simulink model "spherical_wrist"  (R2024b)
settings: Solver=ode23t  StartTime=0.0  StopTime=100  FixedStep=0.001  RelTol=1e-3
InitFcn:
  | WRIST_mk2_1_DataFile
model workspace (MAT data in the model file):
  Damp = Simulink.Parameter
  Damp.Value = 0.0001
  Damp.Complexity = 'real'
  Damp.Dimensions = [1 1]
  Damp.DataType = 'auto'
  Dm = Simulink.Parameter
  Dm.Value = 7.4e-05
  Dm.Complexity = 'real'
  Dm.Dimensions = [1 1]
  Dm.DataType = 'auto'
  Dm.DocUnits = 'mN*m/rpm'
  Jm = Simulink.Parameter
  Jm.Value = 3.3
  Jm.Complexity = 'real'
  Jm.Dimensions = [1 1]
  Jm.DataType = 'auto'
  Jm.DocUnits = 'g*cm^2'
  Km = Simulink.Parameter
  Km.Value = 32.2
  Km.Complexity = 'real'
  Km.Dimensions = [1 1]
  Km.DataType = 'auto'
  Km.DocUnits = 'mN*m/A'
  Tc = Simulink.Parameter
  Tc.Value = 0.001
  Tc.Complexity = 'real'
  Tc.Dimensions = [1 1]
  Tc.DataType = 'auto'
  Tc.DocUnits = 's'
undefined symbols (not defined in the file or in its folder): smiData, X, Y, Z
libraries: sm_lib x370, nesl_utility x32, fl_lib x15, sdl_lib x9, simulink_extras x4, sharedtransform x2, slpidlib x1
(part 1 of 10)
settings Model: Creator=ascalzo  LastModifiedBy=ggandolfi
settings SolverCC: AlgebraicLoopSolver=TrustRegion
settings OptimizationCC: DefaultParameterBehavior=Inlined  UseDivisionForNetSlopeComputation=on  GainParamInheritBuiltInType=on  UseFloatMulNetSlope=on  InlineInvariantSignals=on  ReuseModelBlockBuffer=off  PassReuseOutputArgsAs=Individual arguments  ZeroExternalMemoryAtStartup=off  ZeroInternalMemoryAtStartup=off  NoFixptDivByZeroProtection=on  EfficientFloat2IntCast=on  LifeSpan=1  OptimizeBlockOrder=speed  DifferentSizesBufferReuse=on  EfficientTunableParamExpr=on
settings DebuggingCC: ParameterTunabilityLossMsg=error  UnconnectedInputMsg=warning  UnconnectedOutputMsg=warning  UnconnectedLineMsg=warning
settings HardwareCC: ProdBitPerPointer=32  ProdBitPerSizeT=32  ProdBitPerPtrDiffT=32  ProdLargestAtomicInteger=Long  ProdLargestAtomicFloat=Double  ProdWordSize=32  ProdLongLongMode=on  ProdHWDeviceType=ARM Compatible->ARM Cortex-M
settings ModelReferenceCC: EnableRefExpFcnMdlSchedulingChecks=on
settings SFSimCC: MATLABDynamicMemAlloc=off  SimTargetLang=C++
settings RTWCC: Description=Embedded Coder  SystemTargetFile=ert.tlc  GenCodeOnly=on  PackageGeneratedCodeAndArtifacts=on  PackageName=WristDecoupler.zip  TemplateMakefile=ert_default_tmf  GenerateReport=on  Toolchain=Microsoft Visual C++ 2019 v16.0 | nmake (64-bit Windows)  LaunchReport=on  TargetLang=C++  GPUComputeCapability=3.5  DLArmComputeVersion=19.05
settings CodeAppCC: ForceParamTrailComments=on  IgnoreCustomStorageClasses=off  OperatorAnnotations=on  SimulinkDataObjDesc=on  SFDataObjDesc=on  CustomSymbolStrGlobalVar=rt$N$M  CustomSymbolStrType=$N$M  CustomSymbolStrFcn=$N$M$F  CustomSymbolStrMacro=$N$M  InsertBlockDesc=on  MATLABSourceComments=on
settings ERTTargetCC: TargetLangStandard=C++03 (ISO)  CodeReplacementLibrary=ARM Cortex-M  GenerateSampleERTMain=on  IncludeMdlTerminateFcn=off  CombineSignalStateStructs=on  CodeInterfacePackaging=C++ class  SupportComplex=off  SupportNonInlinedSFcns=on  RootIOFormat=Structure reference  ERTCustomFileTemplate=example_file_process.tlc  ERTFilePackagingFormat=CompactWithDataFile  DynamicArrayContainerType=coder::array
settings ExplorerConfigSet: InternalSimMechanicsExplorerSettings="<ExplorerConfiguration><canonicalview>default</canonicalview><AnimationSetting><BasePlaybackSpeed>1.0</BasePlaybackSpeed><PlaybackSpeedFactor>1.0</PlaybackSpeedFactor></AnimationSetting><TilePanel><TileInfo><Tiles Columns=\"1\" Count=\"1\" Rows=\"1\"><Column Weight=\"1\"/><Row Weight=\"1\"/><Tile Height=\"1\" Width=\"1\" X=\"0\" Y=\"0\"/></Tiles></TileInfo><SceneInfo><SceneViewer><BGColor><R>0.60000002384185791</R><G>0.60000002384185791</G><B>0.60000002384185791</B></BGColor><Camera><DoPerspective>off</DoPerspective><Position><X>0.0033984500914812088</X><Y>-0.99869239330291748</Y><Z>0.0656507387757305771</Z></Position><Center><X>0.0033984500914812088</X><Y>0.00130760669708251953</Y><Z>0.0656507387757305771</Z></Center><Up><X>0</X><Y>-0</Y><Z>1</Z></Up><ViewLimDist>1</ViewLimDist><YLim>0.0676202609390020443</YLim><XLim>0.0894397856975411715</XLim></Camera></SceneViewer></SceneInfo></TilePanel><MechEditorPanel><Cameras/><GfxPanelCameraMap/><VideoCreator><PlaybackSpeedRatio>1.0</PlaybackSpeedRatio><FrameRate>30</FrameRate><VideoFormat>MPEG-4</VideoFormat><FrameSize>[400 400]</FrameSize></VideoCreator></MechEditorPanel></ExplorerConfiguration>"

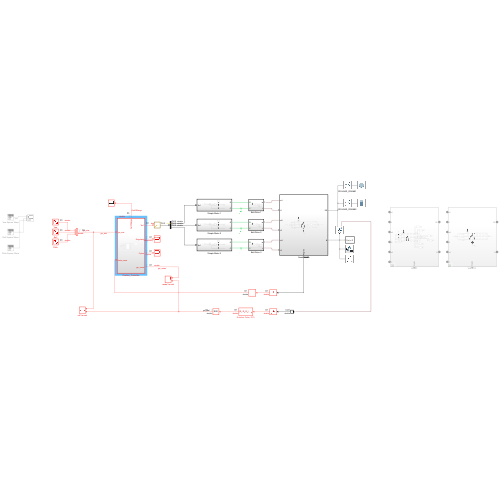
[thumbnail: Simulink's stored preview of the top-level diagram]
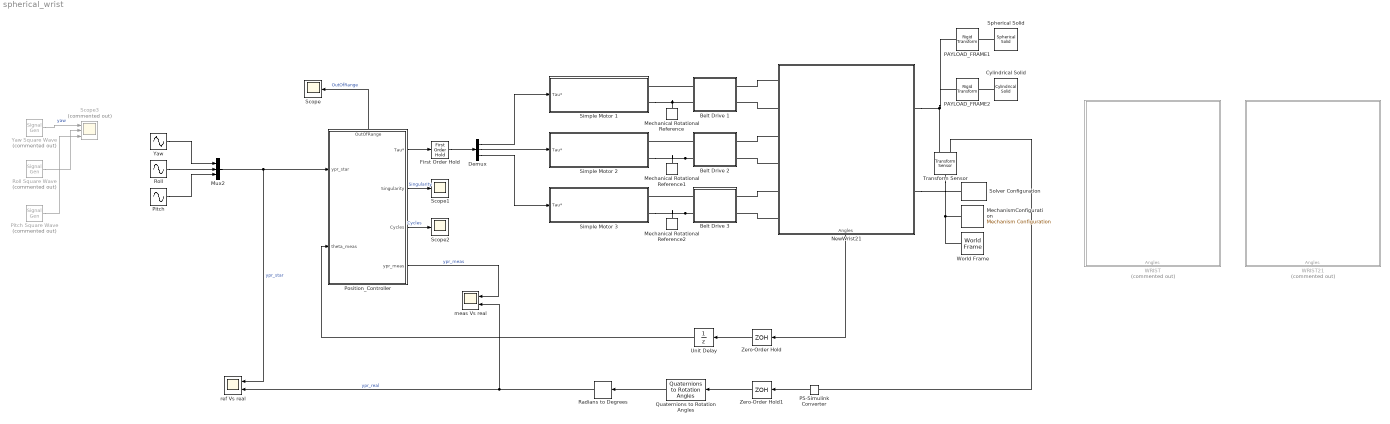
== system spherical_wrist ==
  Belt Drive 1 : Subsystem
  Belt Drive 2 : Subsystem
  Belt Drive 3 : Subsystem
  Cylindrical Solid : sm_lib/Body Elements/Cylindrical Solid  CylinderRadius=4  CylinderRadiusUnits=mm  CylinderLength=56  CylinderLengthUnits=mm  ExportEntireGeometry=off  InertiaType=PointMass  BasedOnType=Density  Density=1000  DensityUnits=kg/m^3  Mass=500  MassUnits=g  CenterOfMass=[0 0 0]  CenterOfMassUnits=m  MomentsOfInertia=[1 1 1]  MomentsOfInertiaUnits=kg*m^2  ProductsOfInertia=[0 0 0]  ProductsOfInertiaUnits=kg*m^2  GraphicType=FromGeometry  MarkerShape=Sphere  MarkerSize=10  GraphicVisPropType=SimpleVisualProperties  GraphicDiffuseColor=[0.5 0.5 0.5]  GraphicOpacity=1  GraphicSpecularColor=[0.5 0.5 0.5 1.0]  GraphicAmbientColor=[0.15 0.15 0.15 1.0]  GraphicEmissiveColor=[0.0 0.0 0.0 1.0]  GraphicShininess=75  DoExposeReferenceFrame=on  SerializedFrames=<Frames/>
  Demux : Demux  Outputs=3
  First Order Hold : FirstOrderHold  ErrorTolerance=inf
  Mechanical Rotational Reference : fl_lib/Mechanical/Rotational Elements/Mechanical Rotational Reference
  Mechanical Rotational Reference1 : fl_lib/Mechanical/Rotational Elements/Mechanical Rotational Reference
  Mechanical Rotational Reference2 : fl_lib/Mechanical/Rotational Elements/Mechanical Rotational Reference
  MechanismConfiguration : sm_lib/Utilities/Mechanism Configuration  UniformGravity=Constant  GravityVector=[0 0 9.80665]  GravityVectorUnits=m/s^2  LinearizationDelta=0.001  JointModeTransitionNonlinearIterations=2
  Mux2 : Mux  Inputs=3
  NewWrist21 : Subsystem
      settings: PortSchema="{\"entries\":[{\"content\":{\"sides\":[{\"content\":{\"connectorIds\":[\"LConn1\",\"LConn2\",\"LConn3\",\"LConn4\",\"LConn5\",\"LConn6\"]},\"type\":\"ConnectorPlacement.EquallySpacedRectSide\",\"uuid\":\"23542f05-d98c-4fd7-a6bd-966b6072cfaf\"},{\"content\":{\"connectorIds\":[\"RConn1\",\"RConn2\"],\"side\":\"RIGHT\"},\"type\":\"ConnectorPlacement.EquallySpacedRectSide\",\"uuid\":\"e7346707-937e-4bb1-b7f6-96a951a5db8c\"},{\"content\":{\"side\":\"TOP\"},\"type\":\"ConnectorPlacement.EquallySpacedRectSide\",\"uuid\":\"63537306-39d7-417a-861f-d22306f14706\"},{\"content\":{\"connectorIds\":[\"Out1\"],\"side\":\"BOTTOM\"},\"type\":\"ConnectorPlacement.EquallySpacedRectSide\",\"uuid\":\"1fb10e15-83ff-4141-85cb-26f173a4368b\"}]},\"type\":\"ConnectorPlacement.EquallySpacedConnector\",\"uuid\":\"ffc830b1-00d2-4766-ad91-ccb75b558bf0\"}],\"packageUris\":[\"http://schema.mathworks.com/mf0/Connector/R2020b\"],\"version\":\"1.0\"}"
  PAYLOAD_FRAME1 : sm_lib/Frames and Transforms/Rigid Transform  RotationMethod=None  FollAlignAxisA=+X  BaseAlignAxisA=+Y  FollAlignAxisB=+Y  BaseAlignAxisB=+Z  RotationStandardAxis=+Z  RotationAngle=smiData.RigidTransform(2).angle  RotationAngleUnits=rad  RotationArbitraryAxis=smiData.RigidTransform(2).axis  RotationSequenceAxes=FollowerAxes  RotationSequence=XYX  RotationSequenceAngles=[0 0 0]  RotationSequenceAnglesUnits=deg  RotationMatrix=[1 0 0; 0 1 0; 0 0 1]  Quaternion=[1 0 0 0]  TranslationMethod=Cartesian  TranslationCartesianOffset=[0 0 70]  TranslationCartesianOffsetUnits=mm  TranslationStandardAxis=+Z  TranslationStandardOffset=0  TranslationStandardOffsetUnits=mm  TranslationROffset=0  TranslationROffsetUnits=m  TranslationThetaOffset=0  TranslationThetaOffsetUnits=deg  TranslationZOffset=0  TranslationZOffsetUnits=m
  PAYLOAD_FRAME2 : sm_lib/Frames and Transforms/Rigid Transform  RotationMethod=None  FollAlignAxisA=+X  BaseAlignAxisA=+Y  FollAlignAxisB=+Y  BaseAlignAxisB=+Z  RotationStandardAxis=+Z  RotationAngle=smiData.RigidTransform(2).angle  RotationAngleUnits=rad  RotationArbitraryAxis=smiData.RigidTransform(2).axis  RotationSequenceAxes=FollowerAxes  RotationSequence=XYX  RotationSequenceAngles=[0 0 0]  RotationSequenceAnglesUnits=deg  RotationMatrix=[1 0 0; 0 1 0; 0 0 1]  Quaternion=[1 0 0 0]  TranslationMethod=Cartesian  TranslationCartesianOffset=[0 0 30]  TranslationCartesianOffsetUnits=mm  TranslationStandardAxis=+Z  TranslationStandardOffset=0  TranslationStandardOffsetUnits=mm  TranslationROffset=0  TranslationROffsetUnits=m  TranslationThetaOffset=0  TranslationThetaOffsetUnits=deg  TranslationZOffset=0  TranslationZOffsetUnits=m
  PS-Simulink Converter : nesl_utility/PS-Simulink Converter  PhysicalDomain=network_engine_domain  SubClassName=ps_output  LeftPortType=input  RightPortType=output  PseudoPeriodic=off  Frequencies=[]  VectorFormat=1-D array  Unit=inherit  AffineConversion=off
  Pitch : Sin  Amplitude=20  Frequency=2*pi/10  SampleTime=Tc
  Pitch Square Wave : SignalGenerator  Commented=on  WaveForm=square  Amplitude=75  Frequency=2*pi/10  Units=rad/sec
  Position_Controller : Subsystem  TreatAsAtomicUnit=on  SystemSampleTime=0.001
      settings: MinAlgLoopOccurrences=on  PortSchema="{\"entries\":[{\"content\":{\"sides\":[{\"content\":{\"connectorIds\":[\"In1\",\"In2\"]},\"type\":\"ConnectorPlacement.EquallySpacedRectSide\",\"uuid\":\"83213a6a-d539-4d4b-893d-998d212c9f51\"},{\"content\":{\"connectorIds\":[\"Out1\",\"Out2\",\"Out3\",\"Out4\"],\"side\":\"RIGHT\"},\"type\":\"ConnectorPlacement.EquallySpacedRectSide\",\"uuid\":\"07d19463-f1b8-4ef2-82ae-a356a5259b0c\"},{\"content\":{\"connectorIds\":[\"Out5\"],\"side\":\"TOP\"},\"type\":\"ConnectorPlacement.EquallySpacedRectSide\",\"uuid\":\"262960f5-5579-40eb-9028-5284e67b897c\"}]},\"type\":\"ConnectorPlacement.EquallySpacedConnector\",\"uuid\":\"3a54d725-4b36-4299-8af9-8f83752d9c8a\"}],\"packageUris\":[\"http://schema.mathworks.com/mf0/Connector/R2020b\"],\"version\":\"1.0\"}"
  Quaternions to Rotation Angles : sharedtransform/Quaternions to Rotation Angles  rotationOrder=ZYX  aMode=aMode
  Radians to Degrees : simulink_extras/Transformations/Radians to Degrees
  Roll : Sin  Amplitude=33  Frequency=(1+sqrt(5))  SampleTime=Tc
  Roll Square Wave : SignalGenerator  Commented=on  WaveForm=square  Amplitude=75  Frequency=(1+sqrt(5))  Units=rad/sec
  Scope : Scope
  Scope1 : Scope
  Scope2 : Scope
  Scope3 : Scope  Commented=on  NumInputPorts=3
  Simple Motor 1 : Subsystem
  Simple Motor 2 : Subsystem
  Simple Motor 3 : Subsystem
  Solver Configuration : nesl_utility/Solver Configuration  PhysicalDomain=network_engine_domain  SubClassName=solver  LeftPortType=input  RightPortType=generic  Tones=[]  Harmonics=[]  SimulateNoise=off  Profile=off  UseLocalSampling=off  EnableSwitchedLinearOptims=on  FrequencyDomain=off  UseCCode=off  RelTol=0.001  AbsTol=1e-06  MinStep=1e-09  ToWorkspace=off  RevertToSquareIcSolve=off  NumHomotopyIterations=100  PhasorMode=off  PhasorModeNumHarmonics=1  ConsistencySolver=NEWTON_FTOL  IndexReductionMethod=DerivativeReplacement  DoDC=off  ResidualTolerance=1e-09  ConsistencyTolSource=GLOBAL  ConsistencyAbsTol=0.001  ConsistencyRelTol=0.001  ConsistencyTolFactor=0.001  UseLocalSolver=off  LocalSolverChoice=NE_TRAPEZOIDAL_ADVANCER  ResolveIndetEquations=on  FunctionEvalNumThread=1  LocalSolverSampleTime=0.0001  DoFixedCost=off  MaxNonlinIter=3  MaxModeIter=2  ComputeImpulses=off  ImpulseIterations=2  LinearAlgebra=auto  LinearAlgebraNumThread=0  EquationFormulation=NE_TIME_EF  DelaysMemoryBudget=1024  AutomaticFiltering=on  FilteringTimeConstant=0.001  PartitionStorageMethod=AS_NEEDED  PartitionMemoryBudget=1024  PartitionMethod=ROBUST  MultibodyUseLocalSolver=off  MultibodyLocalSolverChoice=ODE1  MultibodyLocalSolverSampleTime=0.001
  Spherical Solid : sm_lib/Body Elements/Spherical Solid  SphereRadius=15  SphereRadiusUnits=mm  ExportEntireGeometry=off  InertiaType=CalculateFromGeometry  BasedOnType=Density  Density=1000  DensityUnits=kg/m^3  Mass=1  MassUnits=kg  CenterOfMass=[0 0 0]  CenterOfMassUnits=m  MomentsOfInertia=[1 1 1]  MomentsOfInertiaUnits=kg*m^2  ProductsOfInertia=[0 0 0]  ProductsOfInertiaUnits=kg*m^2  GraphicType=FromGeometry  MarkerShape=Sphere  MarkerSize=10  GraphicVisPropType=SimpleVisualProperties  GraphicDiffuseColor=[0.5 0.5 0.5]  GraphicOpacity=1.0  GraphicSpecularColor=[0.5 0.5 0.5 1.0]  GraphicAmbientColor=[0.15 0.15 0.15 1.0]  GraphicEmissiveColor=[0.0 0.0 0.0 1.0]  GraphicShininess=75  DoExposeReferenceFrame=on  SerializedFrames=<Frames/>
  Transform Sensor : sm_lib/Frames and Transforms/Transform Sensor  MeasurementFrame=World  RotationSequence=XYX  SenseAngle=off  SenseAxis=off  SenseQ=on  SenseR=off  SenseRotationSequence=off  SenseOmegaX=off  SenseOmegaY=off  SenseOmegaZ=off  SenseOmega=off  SenseQDot=off  SenseRDot=off  SenseRotationSequenceDot=off  SenseAlphaX=off  SenseAlphaY=off  SenseAlphaZ=off  SenseAlpha=off  SenseQDDot=off  SenseRDDot=off  SenseX=off  SenseY=off  SenseZ=off  SenseXYZ=off  SenseRad=off  SenseAzim=off  SenseDist=off  SenseInc=off  SenseXDot=off  SenseYDot=off  SenseZDot=off  SenseXYZDot=off  SenseRadDot=off  SenseAzimDot=off  SenseDistDot=off  SenseIncDot=off  SenseXDDot=off  SenseYDDot=off  SenseZDDot=off  SenseXYZDDot=off  SenseRadDDot=off  SenseAzimDDot=off  SenseDistDDot=off  SenseIncDDot=off
  Unit Delay : UnitDelay  SampleTime=-1  HasFrameUpgradeWarning=on
  WRIST : Subsystem  Commented=on
      settings: PortSchema="{\"entries\":[{\"content\":{\"sides\":[{\"content\":{\"connectorIds\":[\"LConn1\",\"LConn2\",\"LConn3\",\"LConn4\",\"LConn5\",\"LConn6\"]},\"type\":\"ConnectorPlacement.EquallySpacedRectSide\",\"uuid\":\"837cba77-e4d8-410a-871c-09f9d5b58985\"},{\"content\":{\"connectorIds\":[\"RConn1\",\"RConn2\"],\"side\":\"RIGHT\"},\"type\":\"ConnectorPlacement.EquallySpacedRectSide\",\"uuid\":\"e99e27fa-5cde-4df4-999c-5c540dbd874f\"},{\"content\":{\"connectorIds\":[],\"side\":\"TOP\"},\"type\":\"ConnectorPlacement.EquallySpacedRectSide\",\"uuid\":\"93dbe70b-6d44-4b10-9b14-70f8e934205d\"},{\"content\":{\"connectorIds\":[\"Out1\"],\"side\":\"BOTTOM\"},\"type\":\"ConnectorPlacement.EquallySpacedRectSide\",\"uuid\":\"bafba6b5-af66-4d82-b4b8-19931a0ab184\"}]},\"type\":\"ConnectorPlacement.EquallySpacedConnector\",\"uuid\":\"c57b24f6-44a7-49b3-8fbc-a4c709c10c31\"}],\"packageUris\":[\"http://schema.mathworks.com/mf0/Connector/19700101\"],\"version\":\"1.0\"}"
  WRIST21 : Subsystem  Commented=on
      settings: PortSchema="{\"entries\":[{\"content\":{\"sides\":[{\"content\":{\"connectorIds\":[\"LConn1\",\"LConn2\",\"LConn3\",\"LConn4\",\"LConn5\",\"LConn6\"]},\"type\":\"ConnectorPlacement.EquallySpacedRectSide\",\"uuid\":\"837cba77-e4d8-410a-871c-09f9d5b58985\"},{\"content\":{\"connectorIds\":[\"RConn1\",\"RConn2\"],\"side\":\"RIGHT\"},\"type\":\"ConnectorPlacement.EquallySpacedRectSide\",\"uuid\":\"e99e27fa-5cde-4df4-999c-5c540dbd874f\"},{\"content\":{\"side\":\"TOP\"},\"type\":\"ConnectorPlacement.EquallySpacedRectSide\",\"uuid\":\"93dbe70b-6d44-4b10-9b14-70f8e934205d\"},{\"content\":{\"connectorIds\":[\"Out1\"],\"side\":\"BOTTOM\"},\"type\":\"ConnectorPlacement.EquallySpacedRectSide\",\"uuid\":\"bafba6b5-af66-4d82-b4b8-19931a0ab184\"}]},\"type\":\"ConnectorPlacement.EquallySpacedConnector\",\"uuid\":\"c57b24f6-44a7-49b3-8fbc-a4c709c10c31\"}],\"packageUris\":[\"http://schema.mathworks.com/mf0/Connector/R2020b\"],\"version\":\"1.0\"}"
  World Frame : sm_lib/Frames and Transforms/World Frame
  Yaw : Sin  Amplitude=92  Frequency=2*pi/40  SampleTime=Tc
  Yaw Square Wave : SignalGenerator  Commented=on  WaveForm=square  Amplitude=90  Frequency=2*pi/40  Units=rad/sec
  Zero-Order Hold : ZeroOrderHold  SampleTime=Tc
  Zero-Order Hold1 : ZeroOrderHold  SampleTime=Tc
  meas Vs real : Scope  NumInputPorts=2
  ref Vs real : Scope  NumInputPorts=2
  wires:
  NewWrist21/1(Angles) -> Zero-Order Hold/1
  Radians to Degrees/1 -> meas Vs real/2, ref Vs real/2  "ypr_real"
  PS-Simulink Converter/1 -> Zero-Order Hold1/1
  Quaternions to Rotation Angles/1 -> Radians to Degrees/1
  Mux2/1 -> Position_Controller/1(ypr_star), ref Vs real/1  "ypr_star"
  Demux/1 -> Simple Motor 1/1(Tau*)
  Demux/2 -> Simple Motor 2/1(Tau*)
  Demux/3 -> Simple Motor 3/1(Tau*)
  First Order Hold/1 -> Demux/1
  Position_Controller/4(ypr_meas) -> meas Vs real/1  "ypr_meas"
  Position_Controller/1(Tau*) -> First Order Hold/1
  Position_Controller/3(Cycles) -> Scope2/1  "Cycles"
  Position_Controller/2(Singularity) -> Scope1/1  "Singularity"
  Zero-Order Hold1/1 -> Quaternions to Rotation Angles/1
  Position_Controller/5(OutOfRange) -> Scope/1  "OutOfRange"
  Zero-Order Hold/1 -> Unit Delay/1
  Roll Square Wave/1 -> Scope3/2
  Pitch Square Wave/1 -> Scope3/3
  Yaw Square Wave/1 -> Scope3/1  "yaw"
  Yaw/1 -> Mux2/1
  Roll/1 -> Mux2/2
  Pitch/1 -> Mux2/3
  Unit Delay/1 -> Position_Controller/2(theta_meas)
  connections:
  World Frame/RConn1 -- NewWrist21/RConn2 -- Transform Sensor/LConn1 -- Solver Configuration/RConn1 -- MechanismConfiguration/RConn1
  PAYLOAD_FRAME1/LConn1 -- PAYLOAD_FRAME2/LConn1 -- NewWrist21/RConn1 -- Transform Sensor/RConn1
  Transform Sensor/RConn2 -- PS-Simulink Converter/LConn1
  Cylindrical Solid/RConn1 -- PAYLOAD_FRAME2/RConn1
  Spherical Solid/RConn1 -- PAYLOAD_FRAME1/RConn1
  NewWrist21/LConn1 -- Belt Drive 1/RConn1
  Mechanical Rotational Reference/LConn1 -- Simple Motor 1/RConn2 -- Belt Drive 1/LConn2
  Belt Drive 1/LConn1 -- Simple Motor 1/RConn1
  Belt Drive 2/LConn2 -- Simple Motor 2/RConn2 -- Mechanical Rotational Reference1/LConn1
  Belt Drive 2/LConn1 -- Simple Motor 2/RConn1
  NewWrist21/LConn3 -- Belt Drive 2/RConn1
  Belt Drive 3/LConn2 -- Simple Motor 3/RConn2 -- Mechanical Rotational Reference2/LConn1
  Belt Drive 3/LConn1 -- Simple Motor 3/RConn1
  NewWrist21/LConn5 -- Belt Drive 3/RConn1
  NewWrist21/LConn2 -- Belt Drive 1/RConn2
  NewWrist21/LConn4 -- Belt Drive 2/RConn2
  NewWrist21/LConn6 -- Belt Drive 3/RConn2

== system spherical_wrist/Belt Drive 1 ==
  Belt Drive : sdl_lib/Couplings & Drives/Belt Drive  drive_type=sdl.enum.wrap_configuration.open  belt_type=sdl.enum.belt_type.ideal  sheave_ang=30 deg  num_belts=1  model_f_c=sdl.enum.model_centrifugal.off  linear_density=0.6 kg/m  model_compliance=sdl.enum.compliance.off  stiffness=1e4 N/m  damping=1e3 N/(m/s)  tension=100 N  breakable=sdl.enum.max_tension.off  F_max=1e5 N  r_pulley_A=14 mm  b_pulley_A=0.1 N*m/(rad/s)  model_inertia_A=sdl.enum.model_inertia.on  pulley_inertia_A=10 g*mm^2  initial_velocity_A=0 rad/s  r_pulley_B=28 mm  b_pulley_B=0.1 N*m/(rad/s)  model_inertia_B=sdl.enum.model_inertia.on  pulley_inertia_B=10 g*mm^2  initial_velocity_B=0 rad/s  friction_model=sdl.enum.PulleyModel.Continuous  initial_state_locked_A=sdl.enum.initial_lock.unlocked  initial_state_locked_B=sdl.enum.initial_lock.unlocked  mu=0.5  mu_static=0.5  mu_kinetic=0.42  wrap_parameterization=sdl.enum.wrap_parameterization.centers  d_centers=0.5 m  phi_wrap_A=145 deg  phi_wrap_B=215 deg  v_thr=0.001 m/s  f_thr=1 N
      settings: InternalSimscapePortConfiguration="{\"Bottom\":[],\"Left\":[{\"id\":\"A\",\"label\":\"A\",\"type\":\"foundation.mechanical.rotational.rotational\"}],\"Right\":[{\"id\":\"B\",\"label\":\"B\",\"type\":\"foundation.mechanical.rotational.rotational\"}],\"Top\":[]}"
  Inertia1 : fl_lib/Mechanical/Rotational Elements/Inertia  inertia=34 g*mm^2  num_ports=foundation.enum.numPorts2.one  w_specify=off  w_priority=High  w=0 rad/s  w_nominal_specify=off  w_nominal_value=1  w_nominal_unit=rad/s  t_specify=off  t_priority=None  t=0 N*m  t_nominal_specify=off  t_nominal_value=1  t_nominal_unit=N*m
  Rotational Multibody Interface : fl_lib/Mechanical/Multibody Interfaces/Rotational Multibody Interface
  Simple Gear : sdl_lib/Gears/Simple Gear  ratio=196  rotation_direction=3-2*(1)  friction_model=sdl.enum.gear_efficiencies_load.constant  T_noload=0.1 N*m  T_nom=5 N*m  efficiency_nom=0.8  efficiency=0.78  temperature_TLU=[280, 300, 320] K  load_TLU=[1, 5, 10] N*m  efficiency_TLU=[.95, .9, .85]  efficiency_TLU2=[.85, .8, .75; .95, .9, .85; .85, .8, .7]  w_thr=0.01 rad/s  pwr_thr=9 W  enable_backlash=false  hardstop_model=simscape.enum.hardstop.smooth  backlash_distance=1e-3 mm  r_base=0.1 m  transition=1e-4 mm  backlash_stiffness=1e7 N/m  backlash_damping=1e6 N*s/m  coeff_rest=0  v_tol=0.001 m/s  f_tol=0 N  mu_visc=[0, 0] N*m/(rad/s)  thermal_mass=50 J/K  temperature_specify=off  temperature_priority=High  temperature=300 K  temperature_nominal_specify=off  temperature_nominal_value=1  temperature_nominal_unit=K  x_backlash_specify=off  x_backlash_priority=None  x_backlash=0 mm  x_backlash_nominal_specify=off  x_backlash_nominal_value=1  x_backlash_nominal_unit=mm  f_hardstop_specify=off  f_hardstop_priority=None  f_hardstop=0 N  f_hardstop_nominal_specify=off  f_hardstop_nominal_value=1  f_hardstop_nominal_unit=N  v_backlash_specify=off  v_backlash_priority=None  v_backlash=0 m/s  v_backlash_nominal_specify=off  v_backlash_nominal_value=1  v_backlash_nominal_unit=m/s
  R : PMIOPort  Side=Left
  C : PMIOPort  Port=2  Side=Left
  w : PMIOPort  Port=3  Side=Right
  t : PMIOPort  Port=4  Side=Right
  connections:
  Rotational Multibody Interface/RConn2 -- Belt Drive/RConn1
  Simple Gear/LConn1 -- R/RConn1 -- Inertia1/LConn1
  Rotational Multibody Interface/RConn1 -- w/RConn1
  Belt Drive/LConn1 -- Simple Gear/RConn1
  Rotational Multibody Interface/LConn1 -- t/RConn1
  Rotational Multibody Interface/LConn2 -- C/RConn1

== system spherical_wrist/Belt Drive 2 ==
  Belt Drive : sdl_lib/Couplings & Drives/Belt Drive  drive_type=sdl.enum.wrap_configuration.open  belt_type=sdl.enum.belt_type.ideal  sheave_ang=30 deg  num_belts=1  model_f_c=sdl.enum.model_centrifugal.off  linear_density=0.6 kg/m  model_compliance=sdl.enum.compliance.off  stiffness=1e4 N/m  damping=1e3 N/(m/s)  tension=100 N  breakable=sdl.enum.max_tension.off  F_max=1e5 N  r_pulley_A=14 mm  b_pulley_A=0.1 N*m/(rad/s)  model_inertia_A=sdl.enum.model_inertia.on  pulley_inertia_A=10 g*mm^2  initial_velocity_A=0 rad/s  r_pulley_B=28 mm  b_pulley_B=0.1 N*m/(rad/s)  model_inertia_B=sdl.enum.model_inertia.on  pulley_inertia_B=10 g*mm^2  initial_velocity_B=0 rad/s  friction_model=sdl.enum.PulleyModel.Continuous  initial_state_locked_A=sdl.enum.initial_lock.unlocked  initial_state_locked_B=sdl.enum.initial_lock.unlocked  mu=0.5  mu_static=0.5  mu_kinetic=0.42  wrap_parameterization=sdl.enum.wrap_parameterization.centers  d_centers=0.5 m  phi_wrap_A=145 deg  phi_wrap_B=215 deg  v_thr=0.001 m/s  f_thr=1 N
      settings: InternalSimscapePortConfiguration="{\"Bottom\":[],\"Left\":[{\"id\":\"A\",\"label\":\"A\",\"type\":\"foundation.mechanical.rotational.rotational\"}],\"Right\":[{\"id\":\"B\",\"label\":\"B\",\"type\":\"foundation.mechanical.rotational.rotational\"}],\"Top\":[]}"
  Inertia1 : fl_lib/Mechanical/Rotational Elements/Inertia  inertia=34 g*mm^2  num_ports=foundation.enum.numPorts2.one  w_specify=off  w_priority=High  w=0 rad/s  w_nominal_specify=off  w_nominal_value=1  w_nominal_unit=rad/s  t_specify=off  t_priority=None  t=0 N*m  t_nominal_specify=off  t_nominal_value=1  t_nominal_unit=N*m
  Rotational Multibody Interface : fl_lib/Mechanical/Multibody Interfaces/Rotational Multibody Interface
  Simple Gear : sdl_lib/Gears/Simple Gear  ratio=196  rotation_direction=3-2*(1)  friction_model=sdl.enum.gear_efficiencies_load.constant  T_noload=0.1 N*m  T_nom=5 N*m  efficiency_nom=0.8  efficiency=0.78  temperature_TLU=[280, 300, 320] K  load_TLU=[1, 5, 10] N*m  efficiency_TLU=[.95, .9, .85]  efficiency_TLU2=[.85, .8, .75; .95, .9, .85; .85, .8, .7]  w_thr=0.01 rad/s  pwr_thr=9 W  enable_backlash=false  hardstop_model=simscape.enum.hardstop.smooth  backlash_distance=1e-3 mm  r_base=0.1 m  transition=1e-4 mm  backlash_stiffness=1e7 N/m  backlash_damping=1e6 N*s/m  coeff_rest=0  v_tol=0.001 m/s  f_tol=0 N  mu_visc=[0, 0] N*m/(rad/s)  thermal_mass=50 J/K  temperature_specify=off  temperature_priority=High  temperature=300 K  temperature_nominal_specify=off  temperature_nominal_value=1  temperature_nominal_unit=K  x_backlash_specify=off  x_backlash_priority=None  x_backlash=0 mm  x_backlash_nominal_specify=off  x_backlash_nominal_value=1  x_backlash_nominal_unit=mm  f_hardstop_specify=off  f_hardstop_priority=None  f_hardstop=0 N  f_hardstop_nominal_specify=off  f_hardstop_nominal_value=1  f_hardstop_nominal_unit=N  v_backlash_specify=off  v_backlash_priority=None  v_backlash=0 m/s  v_backlash_nominal_specify=off  v_backlash_nominal_value=1  v_backlash_nominal_unit=m/s
  R : PMIOPort  Side=Left
  C : PMIOPort  Port=2  Side=Left
  w : PMIOPort  Port=3  Side=Right
  t : PMIOPort  Port=4  Side=Right
  connections:
  Rotational Multibody Interface/RConn2 -- Belt Drive/RConn1
  Inertia1/LConn1 -- Simple Gear/LConn1 -- R/RConn1
  Rotational Multibody Interface/RConn1 -- w/RConn1
  Belt Drive/LConn1 -- Simple Gear/RConn1
  Rotational Multibody Interface/LConn1 -- t/RConn1
  Rotational Multibody Interface/LConn2 -- C/RConn1

== system spherical_wrist/Belt Drive 3 ==
  Belt Drive : sdl_lib/Couplings & Drives/Belt Drive  drive_type=sdl.enum.wrap_configuration.open  belt_type=sdl.enum.belt_type.ideal  sheave_ang=30 deg  num_belts=1  model_f_c=sdl.enum.model_centrifugal.off  linear_density=0.6 kg/m  model_compliance=sdl.enum.compliance.off  stiffness=1e4 N/m  damping=1e3 N/(m/s)  tension=100 N  breakable=sdl.enum.max_tension.off  F_max=1e5 N  r_pulley_A=14 mm  b_pulley_A=0.1 N*m/(rad/s)  model_inertia_A=sdl.enum.model_inertia.on  pulley_inertia_A=10 g*mm^2  initial_velocity_A=0 rad/s  r_pulley_B=28 mm  b_pulley_B=0.1 N*m/(rad/s)  model_inertia_B=sdl.enum.model_inertia.on  pulley_inertia_B=10 g*mm^2  initial_velocity_B=0 rad/s  friction_model=sdl.enum.PulleyModel.Continuous  initial_state_locked_A=sdl.enum.initial_lock.unlocked  initial_state_locked_B=sdl.enum.initial_lock.unlocked  mu=0.5  mu_static=0.5  mu_kinetic=0.42  wrap_parameterization=sdl.enum.wrap_parameterization.centers  d_centers=0.5 m  phi_wrap_A=145 deg  phi_wrap_B=215 deg  v_thr=0.001 m/s  f_thr=1 N
      settings: InternalSimscapePortConfiguration="{\"Bottom\":[],\"Left\":[{\"id\":\"A\",\"label\":\"A\",\"type\":\"foundation.mechanical.rotational.rotational\"}],\"Right\":[{\"id\":\"B\",\"label\":\"B\",\"type\":\"foundation.mechanical.rotational.rotational\"}],\"Top\":[]}"
  Inertia1 : fl_lib/Mechanical/Rotational Elements/Inertia  inertia=34 g*mm^2  num_ports=foundation.enum.numPorts2.one  w_specify=off  w_priority=High  w=0 rad/s  w_nominal_specify=off  w_nominal_value=1  w_nominal_unit=rad/s  t_specify=off  t_priority=None  t=0 N*m  t_nominal_specify=off  t_nominal_value=1  t_nominal_unit=N*m
  Rotational Multibody Interface : fl_lib/Mechanical/Multibody Interfaces/Rotational Multibody Interface
  Simple Gear : sdl_lib/Gears/Simple Gear  ratio=196  rotation_direction=3-2*(1)  friction_model=sdl.enum.gear_efficiencies_load.constant  T_noload=0.1 N*m  T_nom=5 N*m  efficiency_nom=0.8  efficiency=0.78  temperature_TLU=[280, 300, 320] K  load_TLU=[1, 5, 10] N*m  efficiency_TLU=[.95, .9, .85]  efficiency_TLU2=[.85, .8, .75; .95, .9, .85; .85, .8, .7]  w_thr=0.01 rad/s  pwr_thr=9 W  enable_backlash=false  hardstop_model=simscape.enum.hardstop.smooth  backlash_distance=1e-3 mm  r_base=0.1 m  transition=1e-4 mm  backlash_stiffness=1e7 N/m  backlash_damping=1e6 N*s/m  coeff_rest=0  v_tol=0.001 m/s  f_tol=0 N  mu_visc=[0, 0] N*m/(rad/s)  thermal_mass=50 J/K  temperature_specify=off  temperature_priority=High  temperature=300 K  temperature_nominal_specify=off  temperature_nominal_value=1  temperature_nominal_unit=K  x_backlash_specify=off  x_backlash_priority=None  x_backlash=0 mm  x_backlash_nominal_specify=off  x_backlash_nominal_value=1  x_backlash_nominal_unit=mm  f_hardstop_specify=off  f_hardstop_priority=None  f_hardstop=0 N  f_hardstop_nominal_specify=off  f_hardstop_nominal_value=1  f_hardstop_nominal_unit=N  v_backlash_specify=off  v_backlash_priority=None  v_backlash=0 m/s  v_backlash_nominal_specify=off  v_backlash_nominal_value=1  v_backlash_nominal_unit=m/s
  R : PMIOPort  Side=Left
  C : PMIOPort  Port=2  Side=Left
  w : PMIOPort  Port=3  Side=Right
  t : PMIOPort  Port=4  Side=Right
  connections:
  Rotational Multibody Interface/RConn2 -- Belt Drive/RConn1
  Inertia1/LConn1 -- Simple Gear/LConn1 -- R/RConn1
  Rotational Multibody Interface/RConn1 -- w/RConn1
  Belt Drive/LConn1 -- Simple Gear/RConn1
  Rotational Multibody Interface/LConn1 -- t/RConn1
  Rotational Multibody Interface/LConn2 -- C/RConn1

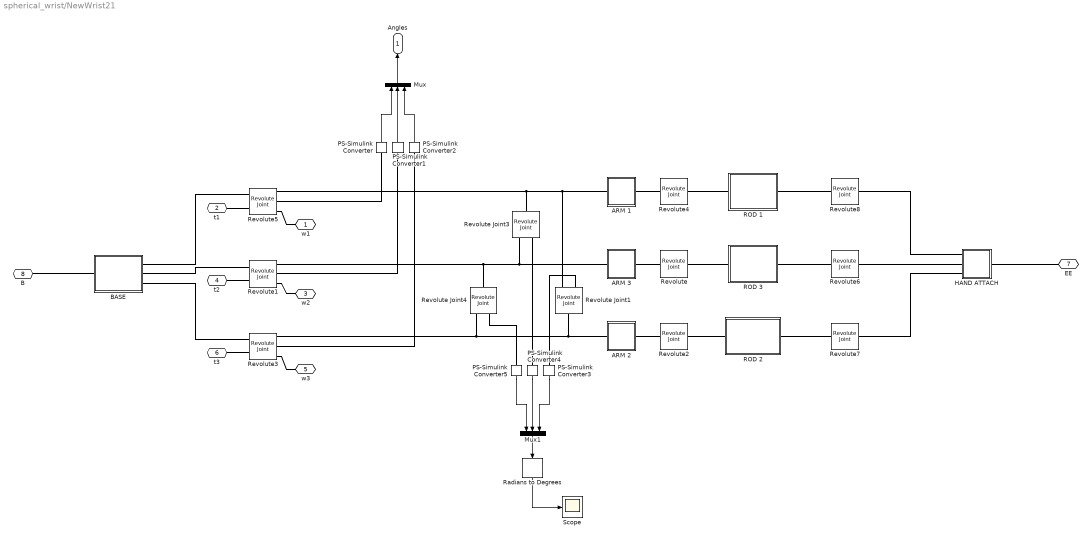
== system spherical_wrist/NewWrist21 ==
  ARM 1 : Subsystem
  ARM 2 : Subsystem
  ARM 3 : Subsystem
  BASE : Subsystem
  HAND ATTACH : Subsystem
  Mux : Mux  Inputs=3
  Mux1 : Mux  Inputs=3
  PS-Simulink Converter : nesl_utility/PS-Simulink Converter  PhysicalDomain=network_engine_domain  SubClassName=ps_output  LeftPortType=input  RightPortType=output  PseudoPeriodic=off  Frequencies=[]  VectorFormat=1-D array  Unit=deg  AffineConversion=off
  PS-Simulink Converter1 : nesl_utility/PS-Simulink Converter  PhysicalDomain=network_engine_domain  SubClassName=ps_output  LeftPortType=input  RightPortType=output  PseudoPeriodic=off  Frequencies=[]  VectorFormat=1-D array  Unit=deg  AffineConversion=off
  PS-Simulink Converter2 : nesl_utility/PS-Simulink Converter  PhysicalDomain=network_engine_domain  SubClassName=ps_output  LeftPortType=input  RightPortType=output  PseudoPeriodic=off  Frequencies=[]  VectorFormat=1-D array  Unit=deg  AffineConversion=off
  PS-Simulink Converter3 : nesl_utility/PS-Simulink Converter  PhysicalDomain=network_engine_domain  SubClassName=ps_output  LeftPortType=input  RightPortType=output  PseudoPeriodic=off  Frequencies=[]  VectorFormat=inherit  Unit=inherit  AffineConversion=off
  PS-Simulink Converter4 : nesl_utility/PS-Simulink Converter  PhysicalDomain=network_engine_domain  SubClassName=ps_output  LeftPortType=input  RightPortType=output  PseudoPeriodic=off  Frequencies=[]  VectorFormat=inherit  Unit=inherit  AffineConversion=off
  PS-Simulink Converter5 : nesl_utility/PS-Simulink Converter  PhysicalDomain=network_engine_domain  SubClassName=ps_output  LeftPortType=input  RightPortType=output  PseudoPeriodic=off  Frequencies=[]  VectorFormat=inherit  Unit=inherit  AffineConversion=off
  ROD 1 : Subsystem
  ROD 2 : Subsystem
  ROD 3 : Subsystem
  Radians to Degrees : simulink_extras/Transformations/Radians to Degrees
  Revolute : sm_lib/Joints/Revolute Joint  JointMode=Normal  CompositeWrenchDir=FollowerOnBase  CompositeWrenchFrame=BaseFrame  SenseConstraintForce=off  SenseConstraintTorque=off  SenseTotalForce=off  SenseTotalTorque=off  PositionTargetSpecify=on  PositionTargetPriority=Low  PositionTargetValue=smiData.RevoluteJoint(1).Rz.Pos  PositionTargetValueUnits=deg  VelocityTargetSpecify=off  VelocityTargetPriority=High  VelocityTargetValue=0  VelocityTargetValueUnits=deg/s  EquilibriumPosition=0  EquilibriumPositionUnits=deg  SpringStiffness=0  SpringStiffnessUnits=N*m/deg  DampingCoefficient=0  DampingCoefficientUnits=N*m/(deg/s)  LowerLimitSpecify=off  LowerLimitBound=-90  LowerLimitBoundUnits=deg  LowerLimitStiffness=1e4  LowerLimitStiffnessUnits=N*m/deg  LowerLimitDamping=10  LowerLimitDampingUnits=N*m/(deg/s)  LowerLimitTransitionRegionWidth=0.1  LowerLimitTransitionRegionWidthUnits=deg  UpperLimitSpecify=off  UpperLimitBound=90  UpperLimitBoundUnits=deg  UpperLimitStiffness=1e4  UpperLimitStiffnessUnits=N*m/deg  UpperLimitDamping=10  UpperLimitDampingUnits=N*m/(deg/s)  UpperLimitTransitionRegionWidth=0.1  UpperLimitTransitionRegionWidthUnits=deg  TorqueActuationMode=NoTorque  MotionActuationMode=ComputedMotion  SensePosition=off  SenseVelocity=off  SenseAcceleration=off  SenseTorqueForce=off  SenseLowerLimitTorqueForce=off  SenseUpperLimitTorqueForce=off
  Revolute Joint1 : sm_lib/Joints/Revolute Joint  JointMode=Normal  CompositeWrenchDir=FollowerOnBase  CompositeWrenchFrame=BaseFrame  SenseConstraintForce=off  SenseConstraintTorque=off  SenseTotalForce=off  SenseTotalTorque=off  PositionTargetSpecify=off  PositionTargetPriority=Low  PositionTargetValue=130  PositionTargetValueUnits=deg  VelocityTargetSpecify=off  VelocityTargetPriority=High  VelocityTargetValue=0  VelocityTargetValueUnits=deg/s  EquilibriumPosition=0  EquilibriumPositionUnits=deg  SpringStiffness=0  SpringStiffnessUnits=N*m/deg  DampingCoefficient=0  DampingCoefficientUnits=N*m/(deg/s)  LowerLimitSpecify=on  LowerLimitBound=33  LowerLimitBoundUnits=deg  LowerLimitStiffness=1e4  LowerLimitStiffnessUnits=N*m/deg  LowerLimitDamping=10  LowerLimitDampingUnits=N*m/(deg/s)  LowerLimitTransitionRegionWidth=0.1  LowerLimitTransitionRegionWidthUnits=deg  UpperLimitSpecify=off  UpperLimitBound=90  UpperLimitBoundUnits=deg  UpperLimitStiffness=1e4  UpperLimitStiffnessUnits=N*m/deg  UpperLimitDamping=10  UpperLimitDampingUnits=N*m/(deg/s)  UpperLimitTransitionRegionWidth=0.1  UpperLimitTransitionRegionWidthUnits=deg  TorqueActuationMode=NoTorque  MotionActuationMode=ComputedMotion  SensePosition=on  SenseVelocity=off  SenseAcceleration=off  SenseTorqueForce=off  SenseLowerLimitTorqueForce=off  SenseUpperLimitTorqueForce=off
  Revolute Joint3 : sm_lib/Joints/Revolute Joint  JointMode=Normal  CompositeWrenchDir=FollowerOnBase  CompositeWrenchFrame=BaseFrame  SenseConstraintForce=off  SenseConstraintTorque=off  SenseTotalForce=off  SenseTotalTorque=off  PositionTargetSpecify=off  PositionTargetPriority=Low  PositionTargetValue=130  PositionTargetValueUnits=deg  VelocityTargetSpecify=off  VelocityTargetPriority=High  VelocityTargetValue=0  VelocityTargetValueUnits=deg/s  EquilibriumPosition=0  EquilibriumPositionUnits=deg  SpringStiffness=0  SpringStiffnessUnits=N*m/deg  DampingCoefficient=0  DampingCoefficientUnits=N*m/(deg/s)  LowerLimitSpecify=on  LowerLimitBound=33  LowerLimitBoundUnits=deg  LowerLimitStiffness=1e4  LowerLimitStiffnessUnits=N*m/deg  LowerLimitDamping=10  LowerLimitDampingUnits=N*m/(deg/s)  LowerLimitTransitionRegionWidth=0.1  LowerLimitTransitionRegionWidthUnits=deg  UpperLimitSpecify=off  UpperLimitBound=90  UpperLimitBoundUnits=deg  UpperLimitStiffness=1e4  UpperLimitStiffnessUnits=N*m/deg  UpperLimitDamping=10  UpperLimitDampingUnits=N*m/(deg/s)  UpperLimitTransitionRegionWidth=0.1  UpperLimitTransitionRegionWidthUnits=deg  TorqueActuationMode=NoTorque  MotionActuationMode=ComputedMotion  SensePosition=on  SenseVelocity=off  SenseAcceleration=off  SenseTorqueForce=off  SenseLowerLimitTorqueForce=off  SenseUpperLimitTorqueForce=off
  Revolute Joint4 : sm_lib/Joints/Revolute Joint  JointMode=Normal  CompositeWrenchDir=FollowerOnBase  CompositeWrenchFrame=BaseFrame  SenseConstraintForce=off  SenseConstraintTorque=off  SenseTotalForce=off  SenseTotalTorque=off  PositionTargetSpecify=off  PositionTargetPriority=Low  PositionTargetValue=130  PositionTargetValueUnits=deg  VelocityTargetSpecify=off  VelocityTargetPriority=High  VelocityTargetValue=0  VelocityTargetValueUnits=deg/s  EquilibriumPosition=0  EquilibriumPositionUnits=deg  SpringStiffness=0  SpringStiffnessUnits=N*m/deg  DampingCoefficient=0  DampingCoefficientUnits=N*m/(deg/s)  LowerLimitSpecify=on  LowerLimitBound=33  LowerLimitBoundUnits=deg  LowerLimitStiffness=1e4  LowerLimitStiffnessUnits=N*m/deg  LowerLimitDamping=10  LowerLimitDampingUnits=N*m/(deg/s)  LowerLimitTransitionRegionWidth=0.1  LowerLimitTransitionRegionWidthUnits=deg  UpperLimitSpecify=off  UpperLimitBound=90  UpperLimitBoundUnits=deg  UpperLimitStiffness=1e4  UpperLimitStiffnessUnits=N*m/deg  UpperLimitDamping=10  UpperLimitDampingUnits=N*m/(deg/s)  UpperLimitTransitionRegionWidth=0.1  UpperLimitTransitionRegionWidthUnits=deg  TorqueActuationMode=NoTorque  MotionActuationMode=ComputedMotion  SensePosition=on  SenseVelocity=off  SenseAcceleration=off  SenseTorqueForce=off  SenseLowerLimitTorqueForce=off  SenseUpperLimitTorqueForce=off
  Revolute1 : sm_lib/Joints/Revolute Joint  JointMode=Normal  CompositeWrenchDir=FollowerOnBase  CompositeWrenchFrame=BaseFrame  SenseConstraintForce=off  SenseConstraintTorque=off  SenseTotalForce=off  SenseTotalTorque=off  PositionTargetSpecify=on  PositionTargetPriority=Low  PositionTargetValue=smiData.RevoluteJoint(2).Rz.Pos  PositionTargetValueUnits=deg  VelocityTargetSpecify=off  VelocityTargetPriority=High  VelocityTargetValue=0  VelocityTargetValueUnits=deg/s  EquilibriumPosition=0  EquilibriumPositionUnits=deg  SpringStiffness=0  SpringStiffnessUnits=N*m/deg  DampingCoefficient=0.001  DampingCoefficientUnits=N*m/(deg/s)  LowerLimitSpecify=off  LowerLimitBound=-90  LowerLimitBoundUnits=deg  LowerLimitStiffness=1e4  LowerLimitStiffnessUnits=N*m/deg  LowerLimitDamping=10  LowerLimitDampingUnits=N*m/(deg/s)  LowerLimitTransitionRegionWidth=0.1  LowerLimitTransitionRegionWidthUnits=deg  UpperLimitSpecify=off  UpperLimitBound=90  UpperLimitBoundUnits=deg  UpperLimitStiffness=1e4  UpperLimitStiffnessUnits=N*m/deg  UpperLimitDamping=10  UpperLimitDampingUnits=N*m/(deg/s)  UpperLimitTransitionRegionWidth=0.1  UpperLimitTransitionRegionWidthUnits=deg  TorqueActuationMode=InputTorque  MotionActuationMode=ComputedMotion  SensePosition=on  SenseVelocity=on  SenseAcceleration=off  SenseTorqueForce=off  SenseLowerLimitTorqueForce=off  SenseUpperLimitTorqueForce=off
  Revolute2 : sm_lib/Joints/Revolute Joint  JointMode=Normal  CompositeWrenchDir=FollowerOnBase  CompositeWrenchFrame=BaseFrame  SenseConstraintForce=off  SenseConstraintTorque=off  SenseTotalForce=off  SenseTotalTorque=off  PositionTargetSpecify=on  PositionTargetPriority=Low  PositionTargetValue=smiData.RevoluteJoint(3).Rz.Pos  PositionTargetValueUnits=deg  VelocityTargetSpecify=off  VelocityTargetPriority=High  VelocityTargetValue=0  VelocityTargetValueUnits=deg/s  EquilibriumPosition=0  EquilibriumPositionUnits=deg  SpringStiffness=0  SpringStiffnessUnits=N*m/deg  DampingCoefficient=0  DampingCoefficientUnits=N*m/(deg/s)  LowerLimitSpecify=off  LowerLimitBound=-90  LowerLimitBoundUnits=deg  LowerLimitStiffness=1e4  LowerLimitStiffnessUnits=N*m/deg  LowerLimitDamping=10  LowerLimitDampingUnits=N*m/(deg/s)  LowerLimitTransitionRegionWidth=0.1  LowerLimitTransitionRegionWidthUnits=deg  UpperLimitSpecify=off  UpperLimitBound=90  UpperLimitBoundUnits=deg  UpperLimitStiffness=1e4  UpperLimitStiffnessUnits=N*m/deg  UpperLimitDamping=10  UpperLimitDampingUnits=N*m/(deg/s)  UpperLimitTransitionRegionWidth=0.1  UpperLimitTransitionRegionWidthUnits=deg  TorqueActuationMode=NoTorque  MotionActuationMode=ComputedMotion  SensePosition=off  SenseVelocity=off  SenseAcceleration=off  SenseTorqueForce=off  SenseLowerLimitTorqueForce=off  SenseUpperLimitTorqueForce=off
  Revolute3 : sm_lib/Joints/Revolute Joint  JointMode=Normal  CompositeWrenchDir=FollowerOnBase  CompositeWrenchFrame=BaseFrame  SenseConstraintForce=off  SenseConstraintTorque=off  SenseTotalForce=off  SenseTotalTorque=off  PositionTargetSpecify=on  PositionTargetPriority=Low  PositionTargetValue=smiData.RevoluteJoint(4).Rz.Pos  PositionTargetValueUnits=deg  VelocityTargetSpecify=off  VelocityTargetPriority=High  VelocityTargetValue=0  VelocityTargetValueUnits=deg/s  EquilibriumPosition=0  EquilibriumPositionUnits=deg  SpringStiffness=0  SpringStiffnessUnits=N*m/deg  DampingCoefficient=0.001  DampingCoefficientUnits=N*m/(deg/s)  LowerLimitSpecify=off  LowerLimitBound=-90  LowerLimitBoundUnits=deg  LowerLimitStiffness=1e4  LowerLimitStiffnessUnits=N*m/deg  LowerLimitDamping=10  LowerLimitDampingUnits=N*m/(deg/s)  LowerLimitTransitionRegionWidth=0.1  LowerLimitTransitionRegionWidthUnits=deg  UpperLimitSpecify=off  UpperLimitBound=90  UpperLimitBoundUnits=deg  UpperLimitStiffness=1e4  UpperLimitStiffnessUnits=N*m/deg  UpperLimitDamping=10  UpperLimitDampingUnits=N*m/(deg/s)  UpperLimitTransitionRegionWidth=0.1  UpperLimitTransitionRegionWidthUnits=deg  TorqueActuationMode=InputTorque  MotionActuationMode=ComputedMotion  SensePosition=on  SenseVelocity=on  SenseAcceleration=off  SenseTorqueForce=off  SenseLowerLimitTorqueForce=off  SenseUpperLimitTorqueForce=off
  Revolute4 : sm_lib/Joints/Revolute Joint  JointMode=Normal  CompositeWrenchDir=FollowerOnBase  CompositeWrenchFrame=BaseFrame  SenseConstraintForce=off  SenseConstraintTorque=off  SenseTotalForce=off  SenseTotalTorque=off  PositionTargetSpecify=on  PositionTargetPriority=Low  PositionTargetValue=smiData.RevoluteJoint(5).Rz.Pos  PositionTargetValueUnits=deg  VelocityTargetSpecify=off  VelocityTargetPriority=High  VelocityTargetValue=0  VelocityTargetValueUnits=deg/s  EquilibriumPosition=0  EquilibriumPositionUnits=deg  SpringStiffness=0  SpringStiffnessUnits=N*m/deg  DampingCoefficient=0  DampingCoefficientUnits=N*m/(deg/s)  LowerLimitSpecify=off  LowerLimitBound=-90  LowerLimitBoundUnits=deg  LowerLimitStiffness=1e4  LowerLimitStiffnessUnits=N*m/deg  LowerLimitDamping=10  LowerLimitDampingUnits=N*m/(deg/s)  LowerLimitTransitionRegionWidth=0.1  LowerLimitTransitionRegionWidthUnits=deg  UpperLimitSpecify=off  UpperLimitBound=90  UpperLimitBoundUnits=deg  UpperLimitStiffness=1e4  UpperLimitStiffnessUnits=N*m/deg  UpperLimitDamping=10  UpperLimitDampingUnits=N*m/(deg/s)  UpperLimitTransitionRegionWidth=0.1  UpperLimitTransitionRegionWidthUnits=deg  TorqueActuationMode=NoTorque  MotionActuationMode=ComputedMotion  SensePosition=off  SenseVelocity=off  SenseAcceleration=off  SenseTorqueForce=off  SenseLowerLimitTorqueForce=off  SenseUpperLimitTorqueForce=off
  Revolute5 : sm_lib/Joints/Revolute Joint  JointMode=Normal  CompositeWrenchDir=FollowerOnBase  CompositeWrenchFrame=BaseFrame  SenseConstraintForce=off  SenseConstraintTorque=off  SenseTotalForce=off  SenseTotalTorque=off  PositionTargetSpecify=on  PositionTargetPriority=Low  PositionTargetValue=smiData.RevoluteJoint(6).Rz.Pos  PositionTargetValueUnits=deg  VelocityTargetSpecify=off  VelocityTargetPriority=High  VelocityTargetValue=0  VelocityTargetValueUnits=deg/s  EquilibriumPosition=0  EquilibriumPositionUnits=deg  SpringStiffness=0  SpringStiffnessUnits=N*m/deg  DampingCoefficient=0.001  DampingCoefficientUnits=N*m/(deg/s)  LowerLimitSpecify=off  LowerLimitBound=-90  LowerLimitBoundUnits=deg  LowerLimitStiffness=1e4  LowerLimitStiffnessUnits=N*m/deg  LowerLimitDamping=10  LowerLimitDampingUnits=N*m/(deg/s)  LowerLimitTransitionRegionWidth=0.1  LowerLimitTransitionRegionWidthUnits=deg  UpperLimitSpecify=off  UpperLimitBound=90  UpperLimitBoundUnits=deg  UpperLimitStiffness=1e4  UpperLimitStiffnessUnits=N*m/deg  UpperLimitDamping=10  UpperLimitDampingUnits=N*m/(deg/s)  UpperLimitTransitionRegionWidth=0.1  UpperLimitTransitionRegionWidthUnits=deg  TorqueActuationMode=InputTorque  MotionActuationMode=ComputedMotion  SensePosition=on  SenseVelocity=on  SenseAcceleration=off  SenseTorqueForce=off  SenseLowerLimitTorqueForce=off  SenseUpperLimitTorqueForce=off
  Revolute6 : sm_lib/Joints/Revolute Joint  JointMode=Normal  CompositeWrenchDir=FollowerOnBase  CompositeWrenchFrame=BaseFrame  SenseConstraintForce=off  SenseConstraintTorque=off  SenseTotalForce=off  SenseTotalTorque=off  PositionTargetSpecify=on  PositionTargetPriority=Low  PositionTargetValue=smiData.RevoluteJoint(7).Rz.Pos  PositionTargetValueUnits=deg  VelocityTargetSpecify=off  VelocityTargetPriority=High  VelocityTargetValue=0  VelocityTargetValueUnits=deg/s  EquilibriumPosition=0  EquilibriumPositionUnits=deg  SpringStiffness=0  SpringStiffnessUnits=N*m/deg  DampingCoefficient=0  DampingCoefficientUnits=N*m/(deg/s)  LowerLimitSpecify=off  LowerLimitBound=-90  LowerLimitBoundUnits=deg  LowerLimitStiffness=1e4  LowerLimitStiffnessUnits=N*m/deg  LowerLimitDamping=10  LowerLimitDampingUnits=N*m/(deg/s)  LowerLimitTransitionRegionWidth=0.1  LowerLimitTransitionRegionWidthUnits=deg  UpperLimitSpecify=off  UpperLimitBound=90  UpperLimitBoundUnits=deg  UpperLimitStiffness=1e4  UpperLimitStiffnessUnits=N*m/deg  UpperLimitDamping=10  UpperLimitDampingUnits=N*m/(deg/s)  UpperLimitTransitionRegionWidth=0.1  UpperLimitTransitionRegionWidthUnits=deg  TorqueActuationMode=NoTorque  MotionActuationMode=ComputedMotion  SensePosition=off  SenseVelocity=off  SenseAcceleration=off  SenseTorqueForce=off  SenseLowerLimitTorqueForce=off  SenseUpperLimitTorqueForce=off
  Revolute7 : sm_lib/Joints/Revolute Joint  JointMode=Normal  CompositeWrenchDir=FollowerOnBase  CompositeWrenchFrame=BaseFrame  SenseConstraintForce=off  SenseConstraintTorque=off  SenseTotalForce=off  SenseTotalTorque=off  PositionTargetSpecify=off  PositionTargetPriority=High  PositionTargetValue=0  PositionTargetValueUnits=deg  VelocityTargetSpecify=off  VelocityTargetPriority=High  VelocityTargetValue=0  VelocityTargetValueUnits=deg/s  EquilibriumPosition=0  EquilibriumPositionUnits=deg  SpringStiffness=0  SpringStiffnessUnits=N*m/deg  DampingCoefficient=0  DampingCoefficientUnits=N*m/(deg/s)  LowerLimitSpecify=off  LowerLimitBound=-90  LowerLimitBoundUnits=deg  LowerLimitStiffness=1e4  LowerLimitStiffnessUnits=N*m/deg  LowerLimitDamping=10  LowerLimitDampingUnits=N*m/(deg/s)  LowerLimitTransitionRegionWidth=0.1  LowerLimitTransitionRegionWidthUnits=deg  UpperLimitSpecify=off  UpperLimitBound=90  UpperLimitBoundUnits=deg  UpperLimitStiffness=1e4  UpperLimitStiffnessUnits=N*m/deg  UpperLimitDamping=10  UpperLimitDampingUnits=N*m/(deg/s)  UpperLimitTransitionRegionWidth=0.1  UpperLimitTransitionRegionWidthUnits=deg  TorqueActuationMode=NoTorque  MotionActuationMode=ComputedMotion  SensePosition=off  SenseVelocity=off  SenseAcceleration=off  SenseTorqueForce=off  SenseLowerLimitTorqueForce=off  SenseUpperLimitTorqueForce=off
  Revolute8 : sm_lib/Joints/Revolute Joint  JointMode=Normal  CompositeWrenchDir=FollowerOnBase  CompositeWrenchFrame=BaseFrame  SenseConstraintForce=off  SenseConstraintTorque=off  SenseTotalForce=off  SenseTotalTorque=off  PositionTargetSpecify=off  PositionTargetPriority=High  PositionTargetValue=0  PositionTargetValueUnits=deg  VelocityTargetSpecify=off  VelocityTargetPriority=High  VelocityTargetValue=0  VelocityTargetValueUnits=deg/s  EquilibriumPosition=0  EquilibriumPositionUnits=deg  SpringStiffness=0  SpringStiffnessUnits=N*m/deg  DampingCoefficient=0  DampingCoefficientUnits=N*m/(deg/s)  LowerLimitSpecify=off  LowerLimitBound=-90  LowerLimitBoundUnits=deg  LowerLimitStiffness=1e4  LowerLimitStiffnessUnits=N*m/deg  LowerLimitDamping=10  LowerLimitDampingUnits=N*m/(deg/s)  LowerLimitTransitionRegionWidth=0.1  LowerLimitTransitionRegionWidthUnits=deg  UpperLimitSpecify=off  UpperLimitBound=90  UpperLimitBoundUnits=deg  UpperLimitStiffness=1e4  UpperLimitStiffnessUnits=N*m/deg  UpperLimitDamping=10  UpperLimitDampingUnits=N*m/(deg/s)  UpperLimitTransitionRegionWidth=0.1  UpperLimitTransitionRegionWidthUnits=deg  TorqueActuationMode=NoTorque  MotionActuationMode=ComputedMotion  SensePosition=off  SenseVelocity=off  SenseAcceleration=off  SenseTorqueForce=off  SenseLowerLimitTorqueForce=off  SenseUpperLimitTorqueForce=off
  Scope : Scope
  w1 : PMIOPort  Side=Left
  t1 : PMIOPort  Port=2  Side=Left
  w2 : PMIOPort  Port=3  Side=Left
  t2 : PMIOPort  Port=4  Side=Left
  w3 : PMIOPort  Port=5  Side=Left
  t3 : PMIOPort  Port=6  Side=Left
  EE : PMIOPort  Port=7  Side=Right
  B : PMIOPort  Port=8  Side=Right
  Angles : Outport
  wires:
  PS-Simulink Converter1/1 -> Mux/2
  PS-Simulink Converter2/1 -> Mux/3
  PS-Simulink Converter/1 -> Mux/1
  Mux/1 -> Angles/1
  PS-Simulink Converter4/1 -> Mux1/2
  PS-Simulink Converter5/1 -> Mux1/1
  PS-Simulink Converter3/1 -> Mux1/3
  Mux1/1 -> Radians to Degrees/1
  Radians to Degrees/1 -> Scope/1
  connections:
  ARM 3/RConn1 -- Revolute/LConn1
  ROD 3/LConn1 -- Revolute/RConn1
  ROD 2/RConn1 -- Revolute7/LConn1
  HAND ATTACH/LConn1 -- Revolute8/RConn1
  HAND ATTACH/LConn3 -- Revolute7/RConn1
  ROD 2/LConn1 -- Revolute2/RConn1
  ARM 2/RConn1 -- Revolute2/LConn1
  ROD 1/RConn1 -- Revolute8/LConn1
  HAND ATTACH/LConn2 -- Revolute6/RConn1
  ROD 3/RConn1 -- Revolute6/LConn1
  ARM 2/LConn1 -- Revolute Joint1/LConn1 -- Revolute Joint4/RConn1 -- Revolute3/RConn1
  BASE/RConn2 -- Revolute1/LConn1
  ARM 3/LConn1 -- Revolute Joint3/RConn1 -- Revolute Joint4/LConn1 -- Revolute1/RConn1
  ARM 1/LConn1 -- Revolute Joint1/RConn1 -- Revolute Joint3/LConn1 -- Revolute5/RConn1
  ARM 1/RConn1 -- Revolute4/LConn1
  ROD 1/LConn1 -- Revolute4/RConn1
  EE/RConn1 -- HAND ATTACH/RConn1
  BASE/RConn1 -- Revolute5/LConn1
  BASE/RConn3 -- Revolute3/LConn1
  B/RConn1 -- BASE/LConn1
  w1/RConn1 -- Revolute5/RConn3
  t1/RConn1 -- Revolute5/LConn2
  t2/RConn1 -- Revolute1/LConn2
  t3/RConn1 -- Revolute3/LConn2
  w2/RConn1 -- Revolute1/RConn3
  w3/RConn1 -- Revolute3/RConn3
  Revolute5/RConn2 -- PS-Simulink Converter/LConn1
  Revolute1/RConn2 -- PS-Simulink Converter1/LConn1
  Revolute3/RConn2 -- PS-Simulink Converter2/LConn1
  Revolute Joint4/RConn2 -- PS-Simulink Converter5/LConn1
  Revolute Joint3/RConn2 -- PS-Simulink Converter4/LConn1
  Revolute Joint1/RConn2 -- PS-Simulink Converter3/LConn1
